simulink model "modelo_miso_compuerta_visual"  (R2026b)
settings: Solver=ode4  StopTime=t_sim  FixedStep=0.001
values from neighbouring files (symbols this model uses):
  b_c = 0.0010    (= 0.001)    [init_parametros.m]
  car_b = 3.5    [init_parametros.m]    (also in polosandzero_car.m)
  car_deadband = 0.005    [init_parametros.m]
  car_F_max = 3.0    (= 3)    [init_parametros.m]    (also in polosandzero_car.m)
  car_Kd = 5    [init_parametros.m]    (also in polosandzero_car.m)
  car_Ki = 10    [init_parametros.m]    (also in polosandzero_car.m)
  car_Kp = 130    [init_parametros.m]
  ctrl_prm = [d0, k_m, m_g*g*l_c, d_min, d_max, pwm_min, pwm_max]    [init_parametros.m]
  d0 = 0.10    (= 0.1)    [init_parametros.m]
  d_ini = d_ini_cm / 100    (= 0.1)    [init_parametros.m]
  d_max = 0.25    [init_parametros.m]
  d_min = 0.05    [init_parametros.m]
  dg_simo = linspace(d_min, d_max, 9)*100    [init_parametros.m]
  fan_dur = 12.0    (= 12)    [init_parametros.m]
  fan_fac = 1.0    (= 1)    [init_parametros.m]
  fan_tau = 0.15    [init_parametros.m]
  g = 9.81    [init_parametros.m]
  gov_deg = 90.0    (= 90)    [init_parametros.m]
  imu_bias = 0.02    [init_parametros.m]
  imu_Ts = 0.01    [init_parametros.m]
  J_g = 0.0002    [init_parametros.m]
  k_m = 0.00030    (= 0.0003)    [init_parametros.m]
  K_pot_deg = V_pot_max / 90.0    (= 0.0183333333333)    [init_parametros.m]
  Kg_simo = zeros(nGs*nDs, 10)    [init_parametros.m]
  l_c = 0.10    (= 0.1)    [init_parametros.m]
  m_car = 0.421    [init_parametros.m]    (also in polosandzero_car.m)
  m_g = 0.015    [init_parametros.m]
  obs_A = A_obs - L_obs*C_obs    [init_parametros.m]
  obs_B = [[1/m_car; 0] - L_obs*D_obs, L_obs]    [init_parametros.m]
  pert_dur = 2.0    (= 2)    [init_parametros.m]
  pert_t_on = 4.0    (= 4)    [init_parametros.m]
  pert_tau_mNm = 0.5    [init_parametros.m]
  pwm_max = 90.0    (= 90)    [init_parametros.m]
  pwm_min = 10.0    (= 10)    [init_parametros.m]
  ref_rate_deg = 200.0    (= 200)    [init_parametros.m]
  sup_prm = [sup_v_hi, sup_v_lo, sup_adv/100, sup_ret/100, d_ini, pwm_min]    [init_parametros.m]
  t_sim = 10.0    (= 10)    [init_parametros.m]
  tau_f = 0.0001    [init_parametros.m]
  tau_ref = 0.15    [init_parametros.m]    (also in simular_sistema.m = 0.45)
  tau_stop = 0.005    [init_parametros.m]
  tau_w = 0.04    [init_parametros.m]
  theta0 = deg2rad(theta0_deg)    [init_parametros.m]
  theta_max = pi/2    (= 1.57079632679)    [init_parametros.m]
  theta_min = 0.0    (= 0)    [init_parametros.m]
  theta_ref_deg = 35.0    (= 35)    [init_parametros.m]
  thg_simo = 10:5:80    [init_parametros.m]
  u_eq0 = min(max(m_g*g*l_c*sin(theta0)/kd_eq, 0), pwm_max)    [init_parametros.m]
  usar_imu = 1    [init_parametros.m]
  V_pot_max = 1.65    [init_parametros.m]
  V_pot_min = 0.0    (= 0)    [init_parametros.m]
  xi_band_deg = 5.0    (= 5)    [init_parametros.m]
  xi_lim = 2.0    (= 2)    [init_parametros.m]
libraries: simulink x6
settings Model: Creator=juane  LastModifiedBy=juane
settings DataIOCC: SaveOutput=off

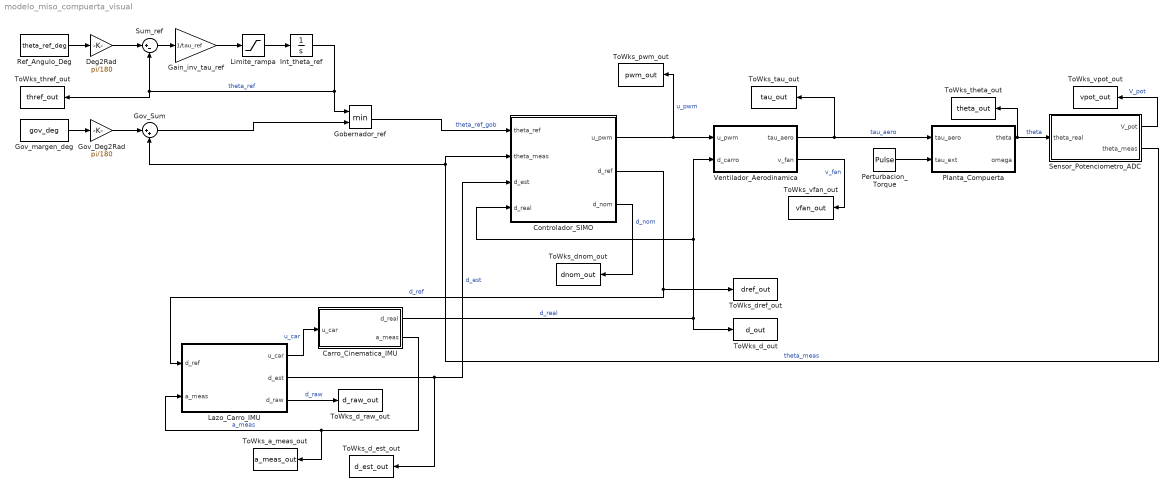
== system modelo_miso_compuerta_visual ==
  Carro_Cinematica_IMU : Subsystem  Description=Subsistema 1/3 (planta): cinematica del carro (masa + friccion), traccion u_car[%] -> d real, y IMU (a_x + sesgo + ruido).
  Controlador_SIMO : Subsystem  Description=Controlador SIMO: entrada theta (ADC) -> salidas u_PWM y d_ref. LQR+I 5 estados con gain scheduling 2-D (theta_ref, d_nom) y supervisor que acerca el carro cuando el ventilador no alcanza.
  Deg2Rad : Gain  Gain=pi/180
  Gain_inv_tau_ref : Gain  Gain=1/tau_ref
  Gobernador_ref : MinMax  Inputs=2
  Gov_Deg2Rad : Gain  Gain=pi/180
  Gov_Sum : Sum  Inputs=|++
  Gov_margen_deg : Constant  Value=gov_deg
  Int_theta_ref : Integrator  InitialCondition=theta0
  Lazo_Carro_IMU : Subsystem  Description=Lazo interno del carro: Kalman de IMU (con entrada F) + PID de posicion con banda muerta.
  Limite_rampa : Saturate  UpperLimit=deg2rad(ref_rate_deg)  LowerLimit=-deg2rad(ref_rate_deg)
  Perturbacion_Torque : DiscretePulseGenerator  PulseType=Time based  Amplitude=pert_tau_mNm*1e-3  Period=2*t_sim  PulseWidth=100*pert_dur/(2*t_sim)  PhaseDelay=pert_t_on
  Planta_Compuerta : Subsystem  Description=Subsistema 3/3 (planta): compuerta colgante de un soporte en L invertida (pendulo, estable). theta = desvio desde el reposo colgante; gravedad restauradora m*g*l*sin(theta). Tope inelastico en 0 y 180 deg.
  Ref_Angulo_Deg : Constant  Value=theta_ref_deg
  Sensor_Potenciometro_ADC : Subsystem
  Sum_ref : Sum  Inputs=|+-
  ToWks_a_meas_out : ToWorkspace  VariableName=a_meas_out  SaveFormat=Timeseries  SampleTime=-1
  ToWks_d_est_out : ToWorkspace  VariableName=d_est_out  SaveFormat=Timeseries  SampleTime=-1
  ToWks_d_out : ToWorkspace  VariableName=d_out  SaveFormat=Timeseries  SampleTime=-1
  ToWks_d_raw_out : ToWorkspace  VariableName=d_raw_out  SaveFormat=Timeseries  SampleTime=-1
  ToWks_dnom_out : ToWorkspace  VariableName=dnom_out  SaveFormat=Timeseries  SampleTime=-1
  ToWks_dref_out : ToWorkspace  VariableName=dref_out  SaveFormat=Timeseries  SampleTime=-1
  ToWks_pwm_out : ToWorkspace  VariableName=pwm_out  SaveFormat=Timeseries  SampleTime=-1
  ToWks_tau_out : ToWorkspace  VariableName=tau_out  SaveFormat=Timeseries  SampleTime=-1
  ToWks_theta_out : ToWorkspace  VariableName=theta_out  SaveFormat=Timeseries  SampleTime=-1
  ToWks_thref_out : ToWorkspace  VariableName=thref_out  SaveFormat=Timeseries  SampleTime=-1
  ToWks_vfan_out : ToWorkspace  VariableName=vfan_out  SaveFormat=Timeseries  SampleTime=-1
  ToWks_vpot_out : ToWorkspace  VariableName=vpot_out  SaveFormat=Timeseries  SampleTime=-1
  Ventilador_Aerodinamica : Subsystem  Description=Subsistema 2/3 (planta): ventilador (lag tau_fan) y torque aerodinamico tau = k_m*f(t)*v_fan*(d0/d)^2, con f(t) = degradacion en rampa del ventilador real (fan_fac).
  wires:
  Ref_Angulo_Deg/1 -> Deg2Rad/1
  Deg2Rad/1 -> Sum_ref/1
  Ventilador_Aerodinamica/1(tau_aero) -> Planta_Compuerta/1(tau_aero), ToWks_tau_out/1  "tau_aero"
  Ventilador_Aerodinamica/2(v_fan) -> ToWks_vfan_out/1  "v_fan"
  Planta_Compuerta/1(theta) -> Sensor_Potenciometro_ADC/1(theta_real), ToWks_theta_out/1  "theta"
  Perturbacion_Torque/1 -> Planta_Compuerta/2(tau_ext)
  Sum_ref/1 -> Gain_inv_tau_ref/1
  Lazo_Carro_IMU/2(d_est) -> Controlador_SIMO/3(d_est), ToWks_d_est_out/1  "d_est"
  Gov_margen_deg/1 -> Gov_Deg2Rad/1
  Gain_inv_tau_ref/1 -> Limite_rampa/1
  Gov_Deg2Rad/1 -> Gov_Sum/1
  Lazo_Carro_IMU/3(d_raw) -> ToWks_d_raw_out/1  "d_raw"
  Sensor_Potenciometro_ADC/1(V_pot) -> ToWks_vpot_out/1  "V_pot"
  Sensor_Potenciometro_ADC/2(theta_meas) -> Gov_Sum/2, Controlador_SIMO/2(theta_meas)  "theta_meas"
  Limite_rampa/1 -> Int_theta_ref/1
  Gov_Sum/1 -> Gobernador_ref/2
  Int_theta_ref/1 -> Gobernador_ref/1, Sum_ref/2, ToWks_thref_out/1  "theta_ref"
  Lazo_Carro_IMU/1(u_car) -> Carro_Cinematica_IMU/1(u_car)  "u_car"
  Gobernador_ref/1 -> Controlador_SIMO/1(theta_ref)  "theta_ref_gob"
  Carro_Cinematica_IMU/1(d_real) -> ToWks_d_out/1, Controlador_SIMO/4(d_real), Ventilador_Aerodinamica/2(d_carro)  "d_real"
  Carro_Cinematica_IMU/2(a_meas) -> ToWks_a_meas_out/1, Lazo_Carro_IMU/2(a_meas)  "a_meas"
  Controlador_SIMO/1(u_pwm) -> Ventilador_Aerodinamica/1(u_pwm), ToWks_pwm_out/1  "u_pwm"
  Controlador_SIMO/2(d_ref) -> Lazo_Carro_IMU/1(d_ref), ToWks_dref_out/1  "d_ref"
  Controlador_SIMO/3(d_nom) -> ToWks_dnom_out/1  "d_nom"

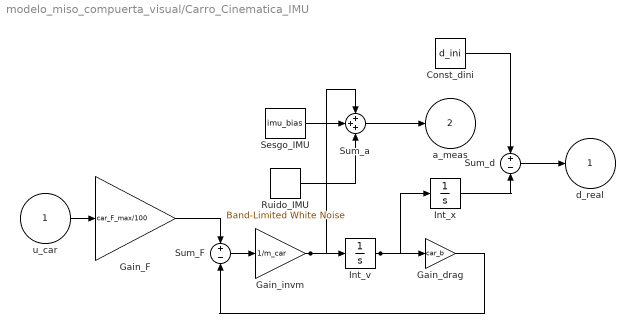
== system modelo_miso_compuerta_visual/Carro_Cinematica_IMU ==
  u_car : Inport
  Const_dini : Constant  Value=d_ini
  Gain_F : Gain  Gain=car_F_max/100
  Gain_drag : Gain  Gain=car_b
  Gain_invm : Gain  Gain=1/m_car
  Int_v : Integrator
  Int_x : Integrator  LimitOutput=on  UpperSaturationLimit=d_ini - d_min  LowerSaturationLimit=d_ini - d_max
  Ruido_IMU : simulink/Sources/Band-Limited White Noise  Cov=imu_noise_pow  Ts=imu_Ts  seed=[42]
  Sesgo_IMU : Constant  Value=imu_bias
  Sum_F : Sum  Inputs=+-
  Sum_a : Sum  Inputs=+++
  Sum_d : Sum  Inputs=+-
  d_real : Outport
  a_meas : Outport  Port=2
  wires:
  Sesgo_IMU/1 -> Sum_a/2
  u_car/1 -> Gain_F/1
  Gain_F/1 -> Sum_F/1
  Gain_invm/1 -> Sum_a/1, Int_v/1
  Sum_F/1 -> Gain_invm/1
  Sum_a/1 -> a_meas/1
  Ruido_IMU/1 -> Sum_a/3
  Int_v/1 -> Gain_drag/1, Int_x/1
  Sum_d/1 -> d_real/1
  Const_dini/1 -> Sum_d/1
  Int_x/1 -> Sum_d/2
  Gain_drag/1 -> Sum_F/2

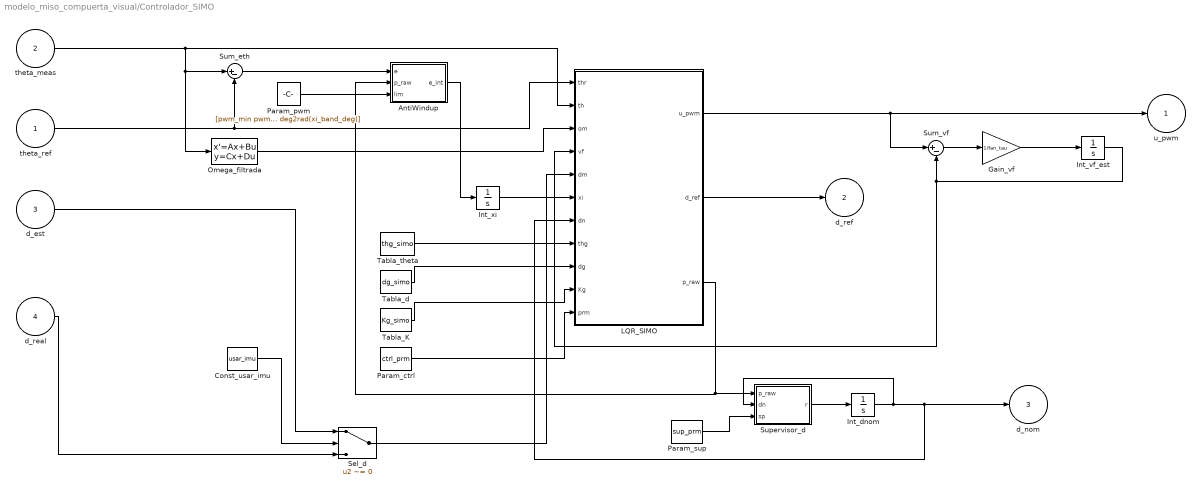
== system modelo_miso_compuerta_visual/Controlador_SIMO ==
  theta_ref : Inport
  theta_meas : Inport  Port=2
  d_est : Inport  Port=3
  d_real : Inport  Port=4
  AntiWindup : MATLAB Function  TreatAsAtomicUnit=on
  Const_usar_imu : Constant  Value=usar_imu
  Gain_vf : Gain  Gain=1/fan_tau
  Int_dnom : Integrator  InitialCondition=d_ini  LimitOutput=on  UpperSaturationLimit=d_max  LowerSaturationLimit=d_min
  Int_vf_est : Integrator  InitialCondition=u_eq0  LimitOutput=on  UpperSaturationLimit=pwm_max  LowerSaturationLimit=0
  Int_xi : Integrator  LimitOutput=on  UpperSaturationLimit=xi_lim  LowerSaturationLimit=-xi_lim
  LQR_SIMO : MATLAB Function  TreatAsAtomicUnit=on
  Omega_filtrada : StateSpace  A=-1/tau_w  B=1/tau_w  C=-1/tau_w  D=1/tau_w  InitialCondition=theta0
  Param_ctrl : Constant  Value=ctrl_prm  VectorParams1D=off
  Param_pwm : Constant  Value=[pwm_min pwm_max deg2rad(xi_band_deg)]  VectorParams1D=off
  Param_sup : Constant  Value=sup_prm  VectorParams1D=off
  Sel_d : Switch  Criteria=u2 ~= 0  SaturateOnIntegerOverflow=off  InputSameDT=off
  Sum_eth : Sum  Inputs=|+-
  Sum_vf : Sum  Inputs=|+-
  Supervisor_d : MATLAB Function  TreatAsAtomicUnit=on
  Tabla_K : Constant  Value=Kg_simo
  Tabla_d : Constant  Value=dg_simo  VectorParams1D=off
  Tabla_theta : Constant  Value=thg_simo  VectorParams1D=off
  u_pwm : Outport
  d_ref : Outport  Port=2
  d_nom : Outport  Port=3
  wires:
  Tabla_K/1 -> LQR_SIMO/10(Kg)
  Supervisor_d/1(r) -> Int_dnom/1
  Sum_eth/1 -> AntiWindup/1(e)
  Tabla_theta/1 -> LQR_SIMO/8(thg)
  Sel_d/1 -> LQR_SIMO/5(dm)
  Sum_vf/1 -> Gain_vf/1
  Param_sup/1 -> Supervisor_d/3(sp)
  theta_meas/1 -> Omega_filtrada/1, Sum_eth/1, LQR_SIMO/2(th)
  d_real/1 -> Sel_d/3
  theta_ref/1 -> LQR_SIMO/1(thr), Sum_eth/2
  d_est/1 -> Sel_d/1
  Const_usar_imu/1 -> Sel_d/2
  Gain_vf/1 -> Int_vf_est/1
  Omega_filtrada/1 -> LQR_SIMO/3(om)
  Int_vf_est/1 -> Sum_vf/2, LQR_SIMO/4(vf)
  Int_dnom/1 -> LQR_SIMO/7(dn), d_nom/1, Supervisor_d/2(dn)
  Tabla_d/1 -> LQR_SIMO/9(dg)
  Param_ctrl/1 -> LQR_SIMO/11(prm)
  LQR_SIMO/1(u_pwm) -> u_pwm/1, Sum_vf/1
  LQR_SIMO/2(d_ref) -> d_ref/1
  LQR_SIMO/3(p_raw) -> AntiWindup/2(p_raw), Supervisor_d/1(p_raw)
  AntiWindup/1(e_int) -> Int_xi/1
  Int_xi/1 -> LQR_SIMO/6(xi)
  Param_pwm/1 -> AntiWindup/3(lim)

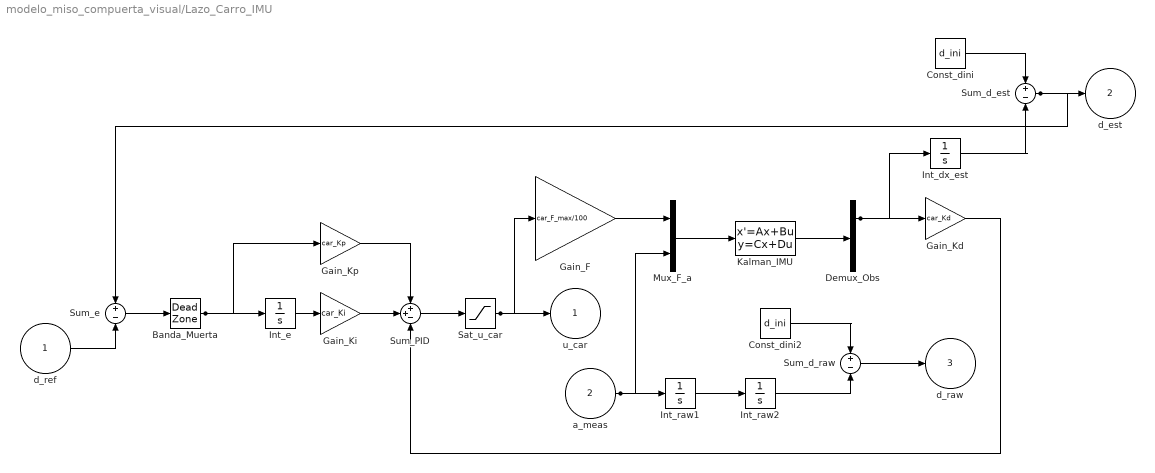
== system modelo_miso_compuerta_visual/Lazo_Carro_IMU ==
  d_ref : Inport
  a_meas : Inport  Port=2
  Banda_Muerta : DeadZone  LowerValue=-car_deadband  UpperValue=car_deadband
  Const_dini : Constant  Value=d_ini
  Const_dini2 : Constant  Value=d_ini
  Demux_Obs : Demux  Outputs=2
  Gain_F : Gain  Gain=car_F_max/100
  Gain_Kd : Gain  Gain=car_Kd
  Gain_Ki : Gain  Gain=car_Ki
  Gain_Kp : Gain  Gain=car_Kp
  Int_dx_est : Integrator
  Int_e : Integrator  LimitOutput=on  UpperSaturationLimit=30/car_Ki  LowerSaturationLimit=-30/car_Ki
  Int_raw1 : Integrator
  Int_raw2 : Integrator
  Kalman_IMU : StateSpace  A=obs_A  B=obs_B  C=eye(2)  D=zeros(2,2)  InitialCondition=[0;0]
  Mux_F_a : Mux  Inputs=2
  Sat_u_car : Saturate  UpperLimit=100  LowerLimit=-100
  Sum_PID : Sum  Inputs=++-
  Sum_d_est : Sum  Inputs=+-
  Sum_d_raw : Sum  Inputs=+-
  Sum_e : Sum  Inputs=+-
  u_car : Outport
  d_est : Outport  Port=2
  d_raw : Outport  Port=3
  wires:
  d_ref/1 -> Sum_e/2
  Gain_Ki/1 -> Sum_PID/2
  Gain_Kp/1 -> Sum_PID/1
  Sum_d_raw/1 -> d_raw/1
  Int_e/1 -> Gain_Ki/1
  Int_raw2/1 -> Sum_d_raw/2
  Banda_Muerta/1 -> Gain_Kp/1, Int_e/1
  Const_dini2/1 -> Sum_d_raw/1
  Sum_e/1 -> Banda_Muerta/1
  Sat_u_car/1 -> u_car/1, Gain_F/1
  Sum_PID/1 -> Sat_u_car/1
  Gain_F/1 -> Mux_F_a/1
  a_meas/1 -> Mux_F_a/2, Int_raw1/1
  Mux_F_a/1 -> Kalman_IMU/1
  Int_raw1/1 -> Int_raw2/1
  Kalman_IMU/1 -> Demux_Obs/1
  Int_dx_est/1 -> Sum_d_est/2
  Demux_Obs/1 -> Gain_Kd/1, Int_dx_est/1
  Sum_d_est/1 -> Sum_e/1, d_est/1
  Const_dini/1 -> Sum_d_est/1
  Gain_Kd/1 -> Sum_PID/3

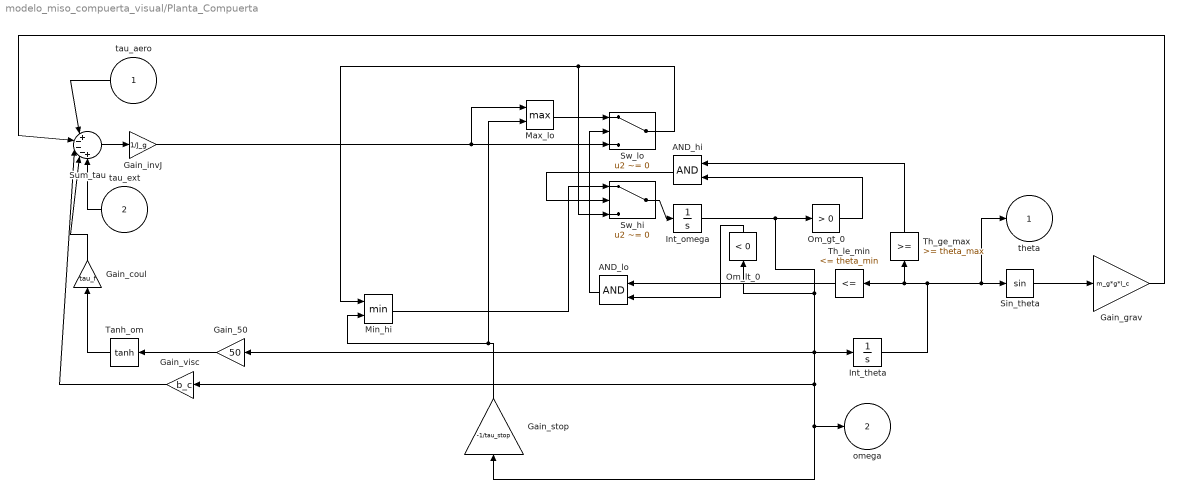
== system modelo_miso_compuerta_visual/Planta_Compuerta ==
  tau_aero : Inport
  tau_ext : Inport  Port=2
  AND_hi : Logic  AllPortsSameDT=off  OutDataTypeStr=boolean
  AND_lo : Logic  AllPortsSameDT=off  OutDataTypeStr=boolean
  Gain_50 : Gain  Gain=50
  Gain_coul : Gain  Gain=tau_f
  Gain_grav : Gain  Gain=m_g*g*l_c
  Gain_invJ : Gain  Gain=1/J_g
  Gain_stop : Gain  Gain=-1/tau_stop
  Gain_visc : Gain  Gain=b_c
  Int_omega : Integrator
  Int_theta : Integrator  InitialCondition=theta0  LimitOutput=on  UpperSaturationLimit=theta_max  LowerSaturationLimit=theta_min
  Max_lo : MinMax  Function=max  Inputs=2
  Min_hi : MinMax  Inputs=2
  Om_gt_0 : simulink/Logic and Bit Operations/Compare To Constant  relop=>  const=0  OutDataTypeStr=boolean
  Om_lt_0 : simulink/Logic and Bit Operations/Compare To Constant  relop=<  const=0  OutDataTypeStr=boolean
  Sin_theta : Trigonometry
  Sum_tau : Sum  Inputs=|+---+
  Sw_hi : Switch  Criteria=u2 ~= 0  SaturateOnIntegerOverflow=off  InputSameDT=off
  Sw_lo : Switch  Criteria=u2 ~= 0  SaturateOnIntegerOverflow=off  InputSameDT=off
  Tanh_om : Trigonometry  Operator=tanh
  Th_ge_max : simulink/Logic and Bit Operations/Compare To Constant  relop=>=  const=theta_max  OutDataTypeStr=boolean
  Th_le_min : simulink/Logic and Bit Operations/Compare To Constant  relop=<=  const=theta_min  OutDataTypeStr=boolean
  theta : Outport
  omega : Outport  Port=2
  wires:
  Int_theta/1 -> theta/1, Sin_theta/1, Th_ge_max/1, Th_le_min/1
  Int_omega/1 -> Int_theta/1, Gain_50/1, Gain_stop/1, omega/1, Gain_visc/1, Om_lt_0/1, Om_gt_0/1
  Gain_50/1 -> Tanh_om/1
  Tanh_om/1 -> Gain_coul/1
  Th_le_min/1 -> AND_lo/1
  Om_lt_0/1 -> AND_lo/2
  Om_gt_0/1 -> AND_hi/2
  Th_ge_max/1 -> AND_hi/1
  Gain_coul/1 -> Sum_tau/4
  Sin_theta/1 -> Gain_grav/1
  tau_aero/1 -> Sum_tau/1
  Gain_grav/1 -> Sum_tau/2
  tau_ext/1 -> Sum_tau/5
  Gain_visc/1 -> Sum_tau/3
  Sum_tau/1 -> Gain_invJ/1
  Gain_invJ/1 -> Sw_lo/3, Max_lo/1
  Gain_stop/1 -> Max_lo/2, Min_hi/2
  Max_lo/1 -> Sw_lo/1
  AND_lo/1 -> Sw_lo/2
  Sw_lo/1 -> Min_hi/1, Sw_hi/3
  Min_hi/1 -> Sw_hi/1
  AND_hi/1 -> Sw_hi/2
  Sw_hi/1 -> Int_omega/1

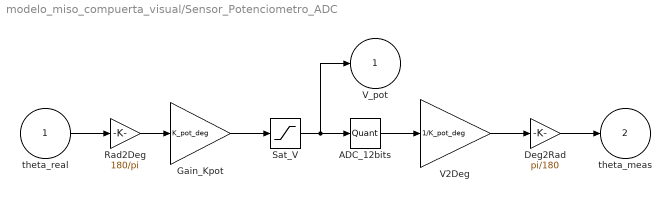
== system modelo_miso_compuerta_visual/Sensor_Potenciometro_ADC ==
  theta_real : Inport
  ADC_12bits : Quantizer  QuantizationInterval=adc_res_V
  Deg2Rad : Gain  Gain=pi/180
  Gain_Kpot : Gain  Gain=K_pot_deg
  Rad2Deg : Gain  Gain=180/pi
  Sat_V : Saturate  UpperLimit=V_pot_max  LowerLimit=V_pot_min
  V2Deg : Gain  Gain=1/K_pot_deg
  V_pot : Outport
  theta_meas : Outport  Port=2
  wires:
  theta_real/1 -> Rad2Deg/1
  Deg2Rad/1 -> theta_meas/1
  V2Deg/1 -> Deg2Rad/1
  ADC_12bits/1 -> V2Deg/1
  Sat_V/1 -> V_pot/1, ADC_12bits/1
  Gain_Kpot/1 -> Sat_V/1
  Rad2Deg/1 -> Gain_Kpot/1

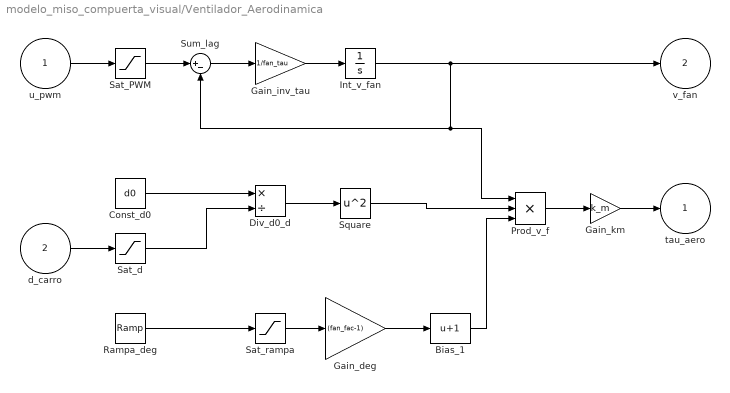
== system modelo_miso_compuerta_visual/Ventilador_Aerodinamica ==
  u_pwm : Inport
  d_carro : Inport  Port=2
  Bias_1 : Bias  Bias=1  SaturateOnIntegerOverflow=off
  Const_d0 : Constant  Value=d0
  Div_d0_d : Product  Inputs=*/
  Gain_deg : Gain  Gain=(fan_fac-1)
  Gain_inv_tau : Gain  Gain=1/fan_tau
  Gain_km : Gain  Gain=k_m
  Int_v_fan : Integrator  InitialCondition=u_eq0  LimitOutput=on  UpperSaturationLimit=pwm_max  LowerSaturationLimit=0
  Prod_v_f : Product  Inputs=***
  Rampa_deg : simulink/Sources/Ramp  slope=1/max(fan_dur,1e-3)  start=fan_t0  InitialOutput=0
  Sat_PWM : Saturate  UpperLimit=pwm_max  LowerLimit=pwm_min
  Sat_d : Saturate  UpperLimit=d_max  LowerLimit=d_min
  Sat_rampa : Saturate  UpperLimit=1  LowerLimit=0
  Square : Math  Operator=square
  Sum_lag : Sum  Inputs=|+-
  tau_aero : Outport
  v_fan : Outport  Port=2
  wires:
  Const_d0/1 -> Div_d0_d/1
  d_carro/1 -> Sat_d/1
  Div_d0_d/1 -> Square/1
  u_pwm/1 -> Sat_PWM/1
  Square/1 -> Prod_v_f/2
  Sat_rampa/1 -> Gain_deg/1
  Sat_d/1 -> Div_d0_d/2
  Bias_1/1 -> Prod_v_f/3
  Gain_deg/1 -> Bias_1/1
  Sum_lag/1 -> Gain_inv_tau/1
  Sat_PWM/1 -> Sum_lag/1
  Rampa_deg/1 -> Sat_rampa/1
  Gain_inv_tau/1 -> Int_v_fan/1
  Int_v_fan/1 -> Prod_v_f/1, Sum_lag/2, v_fan/1
  Prod_v_f/1 -> Gain_km/1
  Gain_km/1 -> tau_aero/1

== matlab function modelo_miso_compuerta_visual/Controlador_SIMO/Supervisor_d ==
  data: p_raw input; r output; dn input; sp input
function r = fcn(p_raw, dn, sp)
% Supervisor de distancia (mueve el punto de operacion d_nom del carro).
% sp = [v_hi, v_lo, v_adv(m/s), v_ret(m/s), d_ini, pwm_min]
% ACERCA si el PWM demandado supera v_hi (el ventilador solo no alcanza / sin margen);
% ALEJA si el PWM demandado cae por debajo del minimo (el ventilador sobra: el minimo ya empuja de mas);
% REGRESA despacio hacia d_ini cuando el PWM queda por debajo de v_lo.
r = 0;
if p_raw > sp(1)
    r = -sp(3) * min(1, (p_raw - sp(1)) / 20);
elseif p_raw < sp(6) - 3
    r = sp(3) * min(1, (sp(6) - 3 - p_raw) / 20);
elseif p_raw < sp(2) && dn < sp(5)
    r = sp(4) * min(1, (sp(2) - p_raw) / 20);
end
end

== matlab function modelo_miso_compuerta_visual/Controlador_SIMO/LQR_SIMO ==
  data: thr input; u_pwm output; th input; om input; vf input; dm input; xi input; dn input; thg input; dg input; Kg input; prm input; d_ref output; p_raw output
function [u_pwm, d_ref, p_raw] = fcn(thr, th, om, vf, dm, xi, dn, thg, dg, Kg, prm)
% LQR+I SIMO con gain scheduling 2-D sobre (theta_ref, d_nom).
% prm = [d0, k_m, m_g*g*l_c, d_min, d_max, pwm_min, pwm_max]; d_nom = punto de operacion de distancia (lo mueve el supervisor)
% x = [th-thr; om; vf-veq; (d-d_nom)*100 [cm]; xi],  u = -K*x = [d_u_PWM; d_d_ref [cm]]
thg = thg(:);  dg = dg(:);
nt = numel(thg);  nd = numel(dg);
thd = min(max(thr*180/pi, thg(1)), thg(nt));
dcm = min(max(dn*100, dg(1)), dg(nd));
i = 1;
for k = 1:nt-1
    if thd >= thg(k)
        i = k;
    end
end
j = 1;
for k = 1:nd-1
    if dcm >= dg(k)
        j = k;
    end
end
wt = (thd - thg(i)) / (thg(i+1) - thg(i));
wd = (dcm - dg(j)) / (dg(j+1) - dg(j));
r11 = (j-1)*nt + i;   r21 = r11 + 1;   r12 = j*nt + i;   r22 = r12 + 1;
Kv = (1-wd)*((1-wt)*Kg(r11,:) + wt*Kg(r21,:)) + wd*((1-wt)*Kg(r12,:) + wt*Kg(r22,:));
K  = reshape(Kv, 2, 5);
veq = prm(3)*sin(thr) / (prm(2)*(prm(1)/dn)^2);
x = [th - thr; om; vf - veq; (dm - dn)*100; xi];
u = -K*x;
p_raw = veq + u(1);
u_pwm = min(max(p_raw, prm(6)), prm(7));
d_ref = min(max(dn + u(2)/100, prm(4)), prm(5));
end

== matlab function modelo_miso_compuerta_visual/Controlador_SIMO/AntiWindup ==
  data: e input; e_int output; p_raw input; lim input
function e_int = fcn(e, p_raw, lim)
% Integra el error theta - theta_ref con dos protecciones (anti-windup):
%  (1) no integra si el PWM esta saturado empujando en esa misma direccion;
%  (2) solo integra con error pequeno (|e| < lim(3)), para no acumular durante la subida rapida.
% lim = [pwm_min, pwm_max, banda_rad]
e_int = e;
if (p_raw >= lim(2) && e < 0) || (p_raw <= lim(1) && e > 0) || abs(e) > lim(3)
    e_int = 0;
end
end
